simulink model "DDMR_Simscape_PID_Motor_2"  (R2024b)
settings: Solver=ode23t  StartTime=0.0  StopTime=60  FixedStep=0.005  RelTol=1e-3
values from neighbouring files (symbols this model uses):
  L = 0.2    [LQR.m]    (also in Track.m; Track2.m)
  L_f = 0.2    [LQR.m]    (also in Track.m; Track2.m)
  line_width = 0.03    [LQR.m]    (also in Track.m; Track2.m)
  N = size(pts, 1)    [Track2.m]
  R = 0.05    [LQR.m]    (also in Track.m; Track2.m)
  track_pts = [2*cos(linspace(0, 2*pi, 1000)'), 2*sin(linspace(0, 2*pi, 1000)').*cos(linspace(0, 2*pi, 1000)')]    [LQR.m]    (also in Track.m; Track2.m = [track_pts; segments{i}])
  W_spread = 0.15    [LQR.m]    (also in Track.m; Track2.m)
undefined symbols (not defined in the file or in its folder): X, Y, Z
libraries: sm_lib x22, fl_lib x8, nesl_utility x8, slpidlib x4, ee_lib x2
(part 2 of 2)

== matlab function DDMR_Simscape_PID_Motor_2/6-Sensor Array1 ==
  data: x input; sensor_readings output; y input; theta input; track_pts input; L_f input; W_spread input; threshold input; sensor_pos output
function [sensor_readings, sensor_pos] = fcn(x, y, theta, track_pts, L_f, W_spread, threshold)
    % 6 sensors spread linearly across the front
    y_offsets = linspace(W_spread/2, -W_spread/2, 6);
    S_loc = [L_f * ones(1,6); y_offsets];
    
    R = [cos(theta), -sin(theta); sin(theta), cos(theta)];
    
    sensor_pos = zeros(2, 6);
    sensor_readings = zeros(1, 6);
    
    for i = 1:6
        % Calculate global position of each sensor
        sensor_pos(:, i) = [x; y] + R * S_loc(:, i);
        
        % Check distance to the track
        dists = sqrt((track_pts(:,1) - sensor_pos(1, i)).^2 + (track_pts(:,2) - sensor_pos(2, i)).^2);
        if min(dists) <= threshold
            sensor_readings(i) = 1;
        end
    end
end

== matlab function DDMR_Simscape_PID_Motor_2/Inverse_Kinematiks 1 ==
  data: v input; omega_L output; omega input; R input; L input; omega_R output
function [omega_L, omega_R] = inverse_kinematics(v, omega, R, L)
    % Calculate linear velocity of each wheel (m/s)
    v_L = v - (omega * L / 2);
    v_R = v + (omega * L / 2);

    % Convert linear velocity to angular velocity (rad/s)
    omega_L = v_L / R;
    omega_R = v_R / R;
end

== matlab function DDMR_Simscape_PID_Motor_2/MATLAB Function1 ==
  settings: updateMethod=DISCRETE
  data: sensor_readings input; e_y output
function e_y = calculate_error(sensor_readings)
    % Physical distances of each sensor from the center of the chassis (in meters)
    % Array total width = 0.15m (+/- 0.075m)
    weights = [0.075, 0.045, 0.015, -0.015, -0.045, -0.075]; 
    
    persistent last_ey
    if isempty(last_ey)
        last_ey = 0;
    end
    
    active_count = sum(sensor_readings);
    
    % Check if BOTH left-wing (1,2) and right-wing (5,6) sensors are lit simultaneously
    both_wings_active = (sensor_readings(1) > 0 || sensor_readings(2) > 0) && ...
                        (sensor_readings(5) > 0 || sensor_readings(6) > 0);
    
    if active_count == 0
        % --- SCENARIO A: All 6 Sensors Read 0 ---
        if abs(last_ey) <= 0.03
            % Robot was centered before losing the line -> DOTTED LINE GAP
            % Output 0 to maintain straight heading across the gap
            e_y = 0;
        else
            % Line slipped off the outer edge (|last_ey| >= 0.045) -> SHARP 90/45/ZIG-ZAG TURN
            % Hold maximum two-sensor error (0.045 + 0.075 = 0.12m) to brake & pivot back
            e_y = sign(last_ey) * 0.12;
        end
        
    elseif both_wings_active || active_count >= 4
        % --- SCENARIO B: 90-Degree Crossroads Intersection ---
        % Perpendicular line triggers sensors across both sides of the array.
        % Ignore the cross-line so the robot drives straight through without twitching.
        e_y = 0;
        last_ey = 0;
        
    else
        % --- SCENARIO C: Normal Line Tracking (Straights, Curves, Zig-Zag, 45-Deg) ---
        % Preserves your exact unnormalized weighted sum
        e_y = sum(sensor_readings .* weights);
        last_ey = e_y;
    end
end
